simulink model "FMT_FlightCore"  (R2026b)
settings: Solver=FixedStepDiscrete  StopTime=26  FixedStep=0.0005
undefined symbols (not defined in the file): CommittedThrust, FlightDiagnostics, fmt_flight_nav_width, NavigationFrame
settings Model: Creator=26718  LastModifiedBy=26718
settings DebuggingCC: AlgebraicLoopMsg=error
settings ModelReferenceCC: ModelReferenceNumInstancesAllowed=Single
settings GRTTargetCC: SubcomponentCodeInterfacePackaging=Nonreusable function

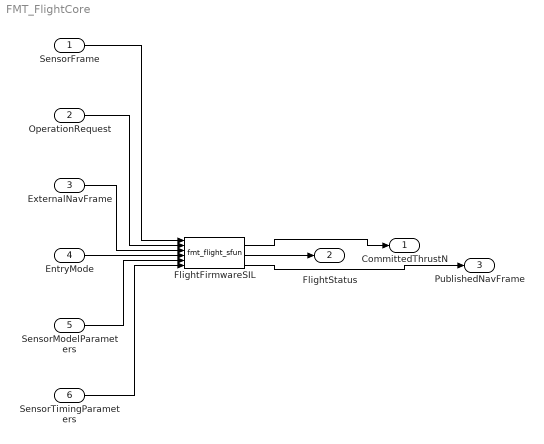
== system FMT_FlightCore ==
  SensorFrame : Inport  OutDataTypeStr=double  PortDimensions=18  SampleTime=0.0005  Interpolate=off
  OperationRequest : Inport  Port=2  OutDataTypeStr=double  PortDimensions=2  SampleTime=0.0005  Interpolate=off
  ExternalNavFrame : Inport  Port=3  OutDataTypeStr=uint8  PortDimensions=fmt_flight_nav_width  SampleTime=0.0005  Interpolate=off
  EntryMode : Inport  Port=4  OutDataTypeStr=double  PortDimensions=1  SampleTime=0.0005  Interpolate=off
  SensorModelParameters : Inport  Port=5  OutDataTypeStr=double  PortDimensions=54  SampleTime=0.0005  Interpolate=off
  SensorTimingParameters : Inport  Port=6  OutDataTypeStr=double  PortDimensions=10  SampleTime=0.0005  Interpolate=off
  FlightFirmwareSIL : S-Function  FunctionName=fmt_flight_sfun  Parameters=fmt_flight_nav_width,fullfile(fileparts(which('fmt_flight_sfun')),'fmt_flight_runtime.dll')  SFunctionDeploymentMode=off  EnableBusSupport=off  SFcnStateName=CommittedThrust,FlightDiagnostics,NavigationFrame
      settings: SFcnIsStateOwnerBlock=on
  CommittedThrustN : Outport
  FlightStatus : Outport  Port=2
  PublishedNavFrame : Outport  Port=3
  wires:
  FlightFirmwareSIL/3 -> PublishedNavFrame/1
  FlightFirmwareSIL/2 -> FlightStatus/1
  FlightFirmwareSIL/1 -> CommittedThrustN/1
  SensorTimingParameters/1 -> FlightFirmwareSIL/6
  SensorModelParameters/1 -> FlightFirmwareSIL/5
  EntryMode/1 -> FlightFirmwareSIL/4
  ExternalNavFrame/1 -> FlightFirmwareSIL/3
  OperationRequest/1 -> FlightFirmwareSIL/2
  SensorFrame/1 -> FlightFirmwareSIL/1
